simulink model "RobustFormationControl_IntegerModel_under_Dis"  (R2023a)
settings: Solver=ode3  StartTime=0.0  StopTime=30  FixedStep=0.0001  RelTol=1e-3
InitFcn:
  | % % Parameters for the fractional order NTFSMC:
  | % Sliding Surface " Sx, Sy, and Sz ":
  | %------------------------
  | % 10
  | % 10
  | cx = 2*[4 4 4];
  | cxx = 1*[0.01 0.01 0.01];
  | 
  | cx1 = cx(1);
  | cy1 = cx(2);
  | cz1 = cx(3);
  | 
  | cx2 = cxx(1);
  | cy2 = cxx(2);
  | cz2 = cxx(3);
  | 
  | alpha1 = [0.6 0.6 0.6];
  | alpha2 = [0.1 0.1 0.1];
  | 
  | gammaX = [3 3 3];
  | gx  = gammaX(1);
  | gy = gammaX(2);
  | gz = gammaX(3);
  | 
  | p = 10;
  | q = 10;
  | 
  | % Sliding Surface " S_Phi , S_Theta, and  S_Psi":
  | %------------------------
  | cP = 2*[4 4 4];
  | cPP = 1*[0.01 0.01 0.01 0.01];
  | 
  | cPhi1 = cP(1);
  | cTheta1 = cP(2);
  | cPsi1 = cP(3);
  | 
  | cPhi2 = cPP(1);
  | cTheta2 = cPP(2);
  | cPsi2 = cPP(3);
  | gammaP = [3 3 3];
  | 
  | %=========================
  | %=========================
  | SigmaX = 1*[0.01 0.01 0.01];
  | SigmaXX =1*[1 1 1];
  | 
  | Sigma1X = SigmaX(1);
  | Sigma1Y = SigmaX(2);
  | Sigma1Z = SigmaX(3);
  | %-----
  | Sigma2X = SigmaXX(1);
  | Sigma2Y = SigmaXX(2);
  | Sigma2Z = SigmaXX(3);
  | 
  | 
  | SigmaP = 1*[0.01 0.01 0.01];
  | SigmaPP =1*[1 1 1];
  | 
  | Sigma1Phi   = SigmaP(1);
  | Sigma1Theta = SigmaP(2);
  | ... (+80 lines)
values from neighbouring files (symbols this model uses):
  a1 = (Iyy - Izz)/Ixx    (= -0.812397034596)    [init_quadrotor_params.m]
  a2 = (Izz - Ixx)/Iyy    (= 0.812397034596)    [init_quadrotor_params.m]
  a3 = (Ixx - Iyy)/Izz    (= 0)    [init_quadrotor_params.m]
  a4 = - Ktx/m    (= -0.00114547325103)    [init_quadrotor_params.m]
  a5 = - Kty/m    (= -0.00114547325103)    [init_quadrotor_params.m]
  a6 = - Ktz/m    (= -0.00130740740741)    [init_quadrotor_params.m]
  b = 2.980e-5    (= 2.98e-05)    [init_quadrotor_params.m]
  b1 = - Jr/Ixx    (= -0.00584534596376)    [init_quadrotor_params.m]
  b2 = Jr/Iyy    (= 0.00584534596376)    [init_quadrotor_params.m]
  b3 = - Kfz/Izz    (= -0.0721963413248)    [init_quadrotor_params.m]
  b4 = 1/m    (= 2.05761316872)    [init_quadrotor_params.m]
  b5 = 1/m    (= 2.05761316872)    [init_quadrotor_params.m]
  b6 = 1/m    (= 2.05761316872)    [init_quadrotor_params.m]
  c1 = - Kfx/Ixx    (= -0.114641680395)    [init_quadrotor_params.m]
  c2 = - Kfy/Iyy    (= -0.114641680395)    [init_quadrotor_params.m]
  c3 = 1/Izz    (= 113.62345188)    [init_quadrotor_params.m]
  d = 1.12e-06    [init_quadrotor_params.m]
  d1 = L/Ixx    (= 46.334431631)    [init_quadrotor_params.m]
  d2 = L/Iyy    (= 46.334431631)    [init_quadrotor_params.m]
  g = 9.81    [init_quadrotor_params.m]
  Ixx = 4.856e-3    (= 0.004856)    [init_quadrotor_params.m]
  Iyy = 4.856e-3    (= 0.004856)    [init_quadrotor_params.m]
  Izz = 8.801e-3    (= 0.008801)    [init_quadrotor_params.m]
  Jr = 2.8385e-5    (= 2.8385e-05)    [init_quadrotor_params.m]
  Kfx = 5.567e-4    (= 0.0005567)    [init_quadrotor_params.m]
  Kfy = 5.567e-4    (= 0.0005567)    [init_quadrotor_params.m]
  Kfz = 6.354e-4    (= 0.0006354)    [init_quadrotor_params.m]
  Ktx = 5.5670e-4    (= 0.0005567)    [init_quadrotor_params.m]
  Kty = 5.5670e-4    (= 0.0005567)    [init_quadrotor_params.m]
  Ktz = 6.3540e-4    (= 0.0006354)    [init_quadrotor_params.m]
  L = 0.225    [init_quadrotor_params.m]
  m = 0.486    [init_quadrotor_params.m]
libraries: fod x120, eeStairGenerator x5
(part 2 of 9)

== system RobustFormationControl_IntegerModel_under_Dis/Integer Leader and four followers/Follower 3 System/ez ==
  note: error analysis for x - position
  note: error analysis for z - position
  note: error analysis for y - position
  e_x : Inport
  e_y : Inport  Port=2
  e_z : Inport  Port=3
  Abs : Abs  SaturateOnIntegerOverflow=off
  Abs1 : Abs  SaturateOnIntegerOverflow=off
  Abs2 : Abs  SaturateOnIntegerOverflow=off
  Clock1 : Clock
  IAE : Display
  IAE1 : Display
  IAE2 : Display
  ISE : Display
  ISE1 : Display
  ISE2 : Display
  ITAE : Display
  ITAE1 : Display
  ITAE2 : Display
  ITSE : Display
  ITSE1 : Display
  ITSE2 : Display
  Integrator{,1..11} (12 alike) : Integrator
  Math Function : Math  Operator=square
  Math Function1 : Math  Operator=square
  Math Function2 : Math  Operator=square
  Mux : Mux
  Mux1 : Mux
  Mux2 : Mux
  Product{,1..5} (6 alike) : Product
  To Workspace : ToWorkspace  VariableName=Ex3  SampleTime=-1
  To Workspace1 : ToWorkspace  VariableName=Ez3  SampleTime=-1
  To Workspace2 : ToWorkspace  VariableName=Ey3  SampleTime=-1
  wires:
  Abs/1 -> Product/1, Integrator/1
  Integrator/1 -> Mux/1, IAE/1
  Math Function/1 -> Product1/1, Integrator1/1
  Integrator1/1 -> Mux/2, ISE/1
  Product/1 -> Integrator2/1
  Integrator2/1 -> Mux/3, ITAE/1
  Product1/1 -> Integrator3/1
  Integrator3/1 -> Mux/4, ITSE/1
  [time] -> Product1/2, Product/2
  [time] -> Product2/2, Product3/2
  Integrator7/1 -> Mux2/4, ITSE1/1
  Product3/1 -> Integrator7/1
  Integrator6/1 -> Mux2/3, ITAE1/1
  Product2/1 -> Integrator6/1
  Integrator5/1 -> Mux2/2, ISE1/1
  Math Function1/1 -> Integrator5/1, Product3/1
  Integrator4/1 -> Mux2/1, IAE1/1
  Abs1/1 -> Integrator4/1, Product2/1
  [ey] -> Abs1/1, Math Function1/1
  [ez] -> Math Function2/1, Abs2/1
  Abs2/1 -> Product4/1, Integrator8/1
  Integrator8/1 -> Mux1/1, IAE2/1
  Math Function2/1 -> Product5/1, Integrator9/1
  Integrator9/1 -> Mux1/2, ISE2/1
  Product4/1 -> Integrator10/1
  Integrator10/1 -> Mux1/3, ITAE2/1
  Product5/1 -> Integrator11/1
  Integrator11/1 -> Mux1/4, ITSE2/1
  [time] -> Product5/2, Product4/2
  e_x/1 -> [ex]
  e_y/1 -> [ey]
  e_z/1 -> [ez]
  Clock1/1 -> [time]
  [ex] -> Math Function/1, Abs/1
  Mux/1 -> To Workspace/1
  Mux1/1 -> To Workspace1/1
  Mux2/1 -> To Workspace2/1

== system RobustFormationControl_IntegerModel_under_Dis/Integer Leader and four followers/Follower 4 System/Desired Values ==
  t : Inport
  Helical Trajectry : Subsystem  Commented=on
  Helical Trajectry1 : Subsystem
  Step : Step  Time=0  After=0.001  SampleTime=0
  Step Inputs Trajectry : Subsystem  Commented=on
  Phi_d : Outport  VectorParamsAs1DForOutWhenUnconnected=off
  Theta_d : Outport  Port=2  VectorParamsAs1DForOutWhenUnconnected=off
  Psi_d : Outport  Port=3  VectorParamsAs1DForOutWhenUnconnected=off
  Xd : Outport  Port=4  VectorParamsAs1DForOutWhenUnconnected=off
  Yd : Outport  Port=5  VectorParamsAs1DForOutWhenUnconnected=off
  Zd : Outport  Port=6  VectorParamsAs1DForOutWhenUnconnected=off
  wires:
  t/1 -> Helical Trajectry1/1(t), Helical Trajectry/1(t)
  Step/1 -> Theta_d/1, Phi_d/1
  Helical Trajectry1/1(xd) -> Xd/1
  Helical Trajectry1/4(Psi_d) -> Psi_d/1
  Helical Trajectry1/2(yd) -> Yd/1
  Helical Trajectry1/3(zd) -> Zd/1

== system RobustFormationControl_IntegerModel_under_Dis/Integer Leader and four followers/Follower 4 System/Follower 2 Quadrotor Model ==
  xd : Inport
  yd : Inport  Port=2
  zd : Inport  Port=3
  Psi_d : Inport  Port=4
  xLeader : Inport  Port=5
  dXYZ : Inport  Port=6
  Control Module1 : Subsystem
  Quadrotor Dynamic System : Subsystem
  X : Outport  VectorParamsAs1DForOutWhenUnconnected=off
  Y : Outport  Port=2  VectorParamsAs1DForOutWhenUnconnected=off
  Z : Outport  Port=3  VectorParamsAs1DForOutWhenUnconnected=off
  Phi : Outport  Port=4  VectorParamsAs1DForOutWhenUnconnected=off
  Theta : Outport  Port=5  VectorParamsAs1DForOutWhenUnconnected=off
  Psi : Outport  Port=6  VectorParamsAs1DForOutWhenUnconnected=off
  U1 : Outport  Port=7  VectorParamsAs1DForOutWhenUnconnected=off
  U2 : Outport  Port=8  VectorParamsAs1DForOutWhenUnconnected=off
  U3 : Outport  Port=9  VectorParamsAs1DForOutWhenUnconnected=off
  U4 : Outport  Port=10  VectorParamsAs1DForOutWhenUnconnected=off
  Ux : Outport  Port=11  VectorParamsAs1DForOutWhenUnconnected=off
  Uy : Outport  Port=12  VectorParamsAs1DForOutWhenUnconnected=off
  wires:
  Control Module1/5(Ux) -> Ux/1, Quadrotor Dynamic System/5(Ux)  "Ux"
  Quadrotor Dynamic System/2(y = x9) -> [x9], Y/1  "Y"
  Quadrotor Dynamic System/6(Psi) -> [x5], Psi/1  "Psi"
  Control Module1/4(U4) -> U4/1, Quadrotor Dynamic System/4(U4)  "U4"
  Quadrotor Dynamic System/3(z = x11) -> [x11], Z/1  "Z"
  Quadrotor Dynamic System/4(Phi) -> [x1], Phi/1  "Phi"
  Quadrotor Dynamic System/5(Theta) -> [x3], Theta/1  "Theta"
  Quadrotor Dynamic System/1(x = x7) -> [x7], X/1  "X"
  Control Module1/6(Uy) -> Uy/1, Quadrotor Dynamic System/6(Uy)  "Uy"
  Control Module1/1(U1) -> Quadrotor Dynamic System/1(U1), U1/1  "U1"
  Control Module1/2(U2) -> Quadrotor Dynamic System/2(U2), U2/1  "U2"
  Control Module1/3(U3) -> U3/1, Quadrotor Dynamic System/3(U3)  "U3"
  Control Module1/7(Omega) -> Quadrotor Dynamic System/7(Omega)
  Quadrotor Dynamic System/7(x2) -> [x2]
  Quadrotor Dynamic System/12(zdot = x12) -> [x12]
  Quadrotor Dynamic System/11(ydot = x10) -> [x10]
  Quadrotor Dynamic System/10(xdot = x8) -> [x8]
  Quadrotor Dynamic System/9(x6) -> [x6]
  Quadrotor Dynamic System/8(x4) -> [x4]
  [x1] -> Control Module1/1(x1)
  [x2] -> Control Module1/2(x2)
  [x3] -> Control Module1/3(x3)
  [x4] -> Control Module1/4(x4)
  [x5] -> Control Module1/5(x5)
  [x6] -> Control Module1/6(x6)
  [x7] -> Control Module1/7(x7)
  [x8] -> Control Module1/8(x8)
  [x9] -> Control Module1/9(x9)
  [x10] -> Control Module1/10(x10)
  [x11] -> Control Module1/11(x11)
  [x12] -> Control Module1/12(x12)
  xd/1 -> Control Module1/14(" xd")
  yd/1 -> Control Module1/15(yd)
  zd/1 -> Control Module1/16(" zd")
  Psi_d/1 -> Control Module1/13(Psi_d)
  xLeader/1 -> Control Module1/17(xLeader)
  dXYZ/1 -> Control Module1/18(Distance_d)

== system RobustFormationControl_IntegerModel_under_Dis/Integer Leader and four followers/Follower 4 System/Results Plot ==
  note: yL
  xF : Inport
  xL : Inport  Port=2
  Demux : Demux  Outputs=3
  Demux1 : Demux  Outputs=3
  x : Scope  NumInputPorts=2
  y : Scope  NumInputPorts=2
  z : Scope  NumInputPorts=2
  wires:
  xF/1 -> Demux/1
  xL/1 -> Demux1/1
  Demux/1 -> x/1  "xF"
  Demux1/1 -> x/2  "xL"
  Demux/2 -> y/1  "yF"
  Demux1/2 -> y/2
  Demux/3 -> z/1  "zF"
  Demux1/3 -> z/2  "zL"

== system RobustFormationControl_IntegerModel_under_Dis/Integer Leader and four followers/Follower 4 System/ez ==
  note: error analysis for x - position
  note: error analysis for z - position
  note: error analysis for y - position
  e_x : Inport
  e_y : Inport  Port=2
  e_z : Inport  Port=3
  Abs : Abs  SaturateOnIntegerOverflow=off
  Abs1 : Abs  SaturateOnIntegerOverflow=off
  Abs2 : Abs  SaturateOnIntegerOverflow=off
  Clock1 : Clock
  IAE : Display
  IAE1 : Display
  IAE2 : Display
  ISE : Display
  ISE1 : Display
  ISE2 : Display
  ITAE : Display
  ITAE1 : Display
  ITAE2 : Display
  ITSE : Display
  ITSE1 : Display
  ITSE2 : Display
  Integrator{,1..11} (12 alike) : Integrator
  Math Function : Math  Operator=square
  Math Function1 : Math  Operator=square
  Math Function2 : Math  Operator=square
  Mux : Mux
  Mux1 : Mux
  Mux2 : Mux
  Product{,1..5} (6 alike) : Product
  To Workspace : ToWorkspace  VariableName=Ex4  SampleTime=-1
  To Workspace1 : ToWorkspace  VariableName=Ez4  SampleTime=-1
  To Workspace2 : ToWorkspace  VariableName=Ey4  SampleTime=-1
  wires:
  Abs/1 -> Product/1, Integrator/1
  Integrator/1 -> Mux/1, IAE/1
  Math Function/1 -> Product1/1, Integrator1/1
  Integrator1/1 -> Mux/2, ISE/1
  Product/1 -> Integrator2/1
  Integrator2/1 -> Mux/3, ITAE/1
  Product1/1 -> Integrator3/1
  Integrator3/1 -> Mux/4, ITSE/1
  [time] -> Product1/2, Product/2
  [time] -> Product2/2, Product3/2
  Integrator7/1 -> Mux2/4, ITSE1/1
  Product3/1 -> Integrator7/1
  Integrator6/1 -> Mux2/3, ITAE1/1
  Product2/1 -> Integrator6/1
  Integrator5/1 -> Mux2/2, ISE1/1
  Math Function1/1 -> Integrator5/1, Product3/1
  Integrator4/1 -> Mux2/1, IAE1/1
  Abs1/1 -> Integrator4/1, Product2/1
  [ey] -> Abs1/1, Math Function1/1
  [ez] -> Math Function2/1, Abs2/1
  Abs2/1 -> Product4/1, Integrator8/1
  Integrator8/1 -> Mux1/1, IAE2/1
  Math Function2/1 -> Product5/1, Integrator9/1
  Integrator9/1 -> Mux1/2, ISE2/1
  Product4/1 -> Integrator10/1
  Integrator10/1 -> Mux1/3, ITAE2/1
  Product5/1 -> Integrator11/1
  Integrator11/1 -> Mux1/4, ITSE2/1
  [time] -> Product5/2, Product4/2
  e_x/1 -> [ex]
  e_y/1 -> [ey]
  e_z/1 -> [ez]
  Clock1/1 -> [time]
  [ex] -> Math Function/1, Abs/1
  Mux/1 -> To Workspace/1
  Mux1/1 -> To Workspace1/1
  Mux2/1 -> To Workspace2/1

== system RobustFormationControl_IntegerModel_under_Dis/Integer Leader and four followers/Leader System/Desired Values ==
  t : Inport
  Circular Trajectry : Subsystem  Commented=on
  Helical Trajectry : Subsystem
  Step : Step  Time=0  After=0.001  SampleTime=0
  Step Inputs Trajectry : Subsystem  Commented=on
  Phi_d : Outport  VectorParamsAs1DForOutWhenUnconnected=off
  Theta_d : Outport  Port=2  VectorParamsAs1DForOutWhenUnconnected=off
  Psi_d : Outport  Port=3  VectorParamsAs1DForOutWhenUnconnected=off
  Xd : Outport  Port=4  VectorParamsAs1DForOutWhenUnconnected=off
  Yd : Outport  Port=5  VectorParamsAs1DForOutWhenUnconnected=off
  Zd : Outport  Port=6  VectorParamsAs1DForOutWhenUnconnected=off
  wires:
  t/1 -> Circular Trajectry/1(t), Helical Trajectry/1(t)
  Step/1 -> Theta_d/1, Phi_d/1
  Helical Trajectry/3(zd) -> Zd/1
  Helical Trajectry/2(yd) -> Yd/1
  Helical Trajectry/1(xd) -> Xd/1
  Helical Trajectry/4(Psi_d) -> Psi_d/1

== system RobustFormationControl_IntegerModel_under_Dis/Integer Leader and four followers/Leader System/Integer Model ==
  xd : Inport
  yd : Inport  Port=2
  zd : Inport  Port=3
  Psi_d : Inport  Port=4
  Control Module1 : Subsystem
  Quadrotor Dynamic System : Subsystem
  Scope : Scope
  X : Outport  VectorParamsAs1DForOutWhenUnconnected=off
  Y : Outport  Port=2  VectorParamsAs1DForOutWhenUnconnected=off
  Z : Outport  Port=3  VectorParamsAs1DForOutWhenUnconnected=off
  Phi : Outport  Port=4  VectorParamsAs1DForOutWhenUnconnected=off
  Theta : Outport  Port=5  VectorParamsAs1DForOutWhenUnconnected=off
  Psi : Outport  Port=6  VectorParamsAs1DForOutWhenUnconnected=off
  U1 : Outport  Port=7  VectorParamsAs1DForOutWhenUnconnected=off
  U2 : Outport  Port=8  VectorParamsAs1DForOutWhenUnconnected=off
  U3 : Outport  Port=9  VectorParamsAs1DForOutWhenUnconnected=off
  U4 : Outport  Port=10  VectorParamsAs1DForOutWhenUnconnected=off
  Ux : Outport  Port=11  VectorParamsAs1DForOutWhenUnconnected=off
  Uy : Outport  Port=12  VectorParamsAs1DForOutWhenUnconnected=off
  wires:
  Control Module1/5(Ux) -> Ux/1, Quadrotor Dynamic System/5(Ux)  "Ux"
  Quadrotor Dynamic System/2(y = x9) -> [x9], Y/1  "Y"
  Quadrotor Dynamic System/6(Psi) -> [x5], Psi/1  "Psi"
  Control Module1/4(U4) -> U4/1, Quadrotor Dynamic System/4(U4)  "U4"
  Quadrotor Dynamic System/3(z = x11) -> [x11], Z/1  "Z"
  Quadrotor Dynamic System/4(Phi) -> [x1], Scope/1, Phi/1  "Phi"
  Quadrotor Dynamic System/5(Theta) -> [x3], Theta/1  "Theta"
  Quadrotor Dynamic System/1(x = x7) -> [x7], X/1  "X"
  Control Module1/6(Uy) -> Uy/1, Quadrotor Dynamic System/6(Uy)  "Uy"
  Control Module1/1(U1) -> Quadrotor Dynamic System/1(U1), U1/1  "U1"
  Control Module1/2(U2) -> Quadrotor Dynamic System/2(U2), U2/1  "U2"
  Control Module1/3(U3) -> U3/1, Quadrotor Dynamic System/3(U3)  "U3"
  Control Module1/7(Omega) -> Quadrotor Dynamic System/7(Omega)
  Quadrotor Dynamic System/7(x2) -> [x2]
  Quadrotor Dynamic System/12(zdot = x12) -> [x12]
  Quadrotor Dynamic System/11(ydot = x10) -> [x10]
  Quadrotor Dynamic System/10(xdot = x8) -> [x8]
  Quadrotor Dynamic System/9(x6) -> [x6]
  Quadrotor Dynamic System/8(x4) -> [x4]
  [x1] -> Control Module1/1(x1)
  [x2] -> Control Module1/2(x2)
  [x3] -> Control Module1/3(x3)
  [x4] -> Control Module1/4(x4)
  [x5] -> Control Module1/5(x5)
  [x6] -> Control Module1/6(x6)
  [x7] -> Control Module1/7(x7)
  [x8] -> Control Module1/8(x8)
  [x9] -> Control Module1/9(x9)
  [x10] -> Control Module1/10(x10)
  [x11] -> Control Module1/11(x11)
  [x12] -> Control Module1/12(x12)
  xd/1 -> Control Module1/14(" xd")
  yd/1 -> Control Module1/15(yd)
  zd/1 -> Control Module1/16(" zd")
  Psi_d/1 -> Control Module1/13(Psi_d)

== system RobustFormationControl_IntegerModel_under_Dis/Integer Leader and four followers/Leader System/Stochastic Disturbances ==
  Dphi1 : Subsystem
  Dphi2 : Subsystem
  Dphi3 : Subsystem
  Dpx : Subsystem
  Dpy : Subsystem
  Dpz : Subsystem
  Mux : Mux  Inputs=3
  Mux1 : Mux  Inputs=3
  To Workspace : ToWorkspace  VariableName=DisP  SampleTime=-1
  To Workspace1 : ToWorkspace  VariableName=DisA  SampleTime=-1
  tag scope: Dphi1=global, Dphi2=global, Dphi3=global, Dpx=global, Dpy=global, Dpz=global
  wires:
  Dpx/1(Dpx) -> [Dpx]
  Dpy/1(Dpy) -> [Dpy]
  Dpz/1(Dpz) -> [Dpz]
  Dphi1/1(Dphi1) -> [Dphi1]
  Dphi2/1(Dphi2) -> [Dphi2]
  Dphi3/1(Dphi3) -> [Dphi3]
  Mux/1 -> To Workspace/1
  Mux1/1 -> To Workspace1/1
  [Dpx] -> Mux/1
  [Dpy] -> Mux/2
  [Dpz] -> Mux/3
  [Dphi1] -> Mux1/1
  [Dphi2] -> Mux1/2
  [Dphi3] -> Mux1/3

== system RobustFormationControl_IntegerModel_under_Dis/Integer Leader and four followers/Leader System/Uncertainity ==
  uncertainity in mass : Subsystem
  uncertainity in moments of inertia : Subsystem

== system RobustFormationControl_IntegerModel_under_Dis/Integer Leader and four followers/Leader System/ez ==
  note: error analysis for x - position
  note: error analysis for z - position
  note: error analysis for y - position
  e_x : Inport
  e_y : Inport  Port=2
  e_z : Inport  Port=3
  Abs : Abs  SaturateOnIntegerOverflow=off
  Abs1 : Abs  SaturateOnIntegerOverflow=off
  Abs2 : Abs  SaturateOnIntegerOverflow=off
  Clock1 : Clock
  IAE : Display
  IAE1 : Display
  IAE2 : Display
  ISE : Display
  ISE1 : Display
  ISE2 : Display
  ITAE : Display
  ITAE1 : Display
  ITAE2 : Display
  ITSE : Display
  ITSE1 : Display
  ITSE2 : Display
  Integrator{,1..11} (12 alike) : Integrator
  Math Function : Math  Operator=square
  Math Function1 : Math  Operator=square
  Math Function2 : Math  Operator=square
  Mux : Mux
  Mux1 : Mux
  Mux2 : Mux
  Product{,1..5} (6 alike) : Product
  To Workspace : ToWorkspace  VariableName=Ex  SampleTime=-1
  To Workspace1 : ToWorkspace  VariableName=Ez  SampleTime=-1
  To Workspace2 : ToWorkspace  VariableName=Ey  SampleTime=-1
  wires:
  Abs/1 -> Product/1, Integrator/1
  Integrator/1 -> Mux/1, IAE/1
  Math Function/1 -> Product1/1, Integrator1/1
  Integrator1/1 -> Mux/2, ISE/1
  Product/1 -> Integrator2/1
  Integrator2/1 -> Mux/3, ITAE/1
  Product1/1 -> Integrator3/1
  Integrator3/1 -> Mux/4, ITSE/1
  [time] -> Product1/2, Product/2
  [time] -> Product2/2, Product3/2
  Integrator7/1 -> Mux2/4, ITSE1/1
  Product3/1 -> Integrator7/1
  Integrator6/1 -> Mux2/3, ITAE1/1
  Product2/1 -> Integrator6/1
  Integrator5/1 -> Mux2/2, ISE1/1
  Math Function1/1 -> Integrator5/1, Product3/1
  Integrator4/1 -> Mux2/1, IAE1/1
  Abs1/1 -> Integrator4/1, Product2/1
  [ey] -> Abs1/1, Math Function1/1
  [ez] -> Math Function2/1, Abs2/1
  Abs2/1 -> Product4/1, Integrator8/1
  Integrator8/1 -> Mux1/1, IAE2/1
  Math Function2/1 -> Product5/1, Integrator9/1
  Integrator9/1 -> Mux1/2, ISE2/1
  Product4/1 -> Integrator10/1
  Integrator10/1 -> Mux1/3, ITAE2/1
  Product5/1 -> Integrator11/1
  Integrator11/1 -> Mux1/4, ITSE2/1
  [time] -> Product5/2, Product4/2
  e_x/1 -> [ex]
  e_y/1 -> [ey]
  e_z/1 -> [ez]
  Clock1/1 -> [time]
  [ex] -> Math Function/1, Abs/1
  Mux/1 -> To Workspace/1
  Mux1/1 -> To Workspace1/1
  Mux2/1 -> To Workspace2/1

== system RobustFormationControl_IntegerModel_under_Dis/Integer Leader and four followers/Follower 1 System/Desired Values/Helical Trajectry ==
  t : Inport
  Gain2 : Gain  Gain=0.2
  Step1 : Step  Time=0  SampleTime=0
  Trigonometric Function : Trigonometry
  Trigonometric Function1 : Trigonometry  Operator=cos
  xd : Outport  VectorParamsAs1DForOutWhenUnconnected=off
  yd : Outport  Port=2  VectorParamsAs1DForOutWhenUnconnected=off
  zd : Outport  Port=3  VectorParamsAs1DForOutWhenUnconnected=off
  Psi_d : Outport  Port=4  VectorParamsAs1DForOutWhenUnconnected=off
  wires:
  t/1 -> Trigonometric Function1/1, Trigonometric Function/1, Gain2/1
  Gain2/1 -> zd/1
  Step1/1 -> Psi_d/1
  Trigonometric Function1/1 -> xd/1
  Trigonometric Function/1 -> yd/1

== system RobustFormationControl_IntegerModel_under_Dis/Integer Leader and four followers/Follower 1 System/Desired Values/Helical Trajectry1 ==
  t : Inport
  Gain : Gain  Gain=dis
  Gain1 : Gain  Gain=2*pi/15
  Gain2 : Gain  Gain=1/15
  Gain3 : Gain  Gain=2*pi/15
  Scope : Scope
  Step : Step  Time=0  After=0  SampleTime=0.03
  Step1 : Step  Time=0  SampleTime=0
  Step2 : Step  Time=5  After=0.5  SampleTime=0.03
  Step3 : Step  Time=10  After=0.5  SampleTime=0.03
  Sum : Sum  Inputs=++-
  Sum1 : Sum  Inputs=|++
  Trigonometric Function : Trigonometry  Operator=cos
  Trigonometric Function1 : Trigonometry
  xd : Outport  VectorParamsAs1DForOutWhenUnconnected=off
  yd : Outport  Port=2  VectorParamsAs1DForOutWhenUnconnected=off
  zd : Outport  Port=3  VectorParamsAs1DForOutWhenUnconnected=off
  Psi_d : Outport  Port=4  VectorParamsAs1DForOutWhenUnconnected=off
  wires:
  t/1 -> Gain1/1, Gain3/1, Gain2/1
  Gain2/1 -> zd/1
  Step1/1 -> Psi_d/1
  Trigonometric Function1/1 -> yd/1
  Step/1 -> Sum/1
  Sum/1 -> Gain/1, Scope/1
  Step2/1 -> Sum/2
  Step3/1 -> Sum/3
  Sum1/1 -> xd/1
  Trigonometric Function/1 -> Sum1/2
  Gain/1 -> Sum1/1
  Gain1/1 -> Trigonometric Function/1
  Gain3/1 -> Trigonometric Function1/1

== system RobustFormationControl_IntegerModel_under_Dis/Integer Leader and four followers/Follower 1 System/Desired Values/Step Inputs Trajectry ==
  Step : Step  Time=0  After=3  SampleTime=0
  Step1 : Step  Time=0  After=5  SampleTime=0
  Step2 : Step  Time=0  SampleTime=0
  Step3 : Step  Time=0  After=2  SampleTime=0
  xd : Outport  VectorParamsAs1DForOutWhenUnconnected=off
  yd : Outport  Port=2  VectorParamsAs1DForOutWhenUnconnected=off
  zd : Outport  Port=3  VectorParamsAs1DForOutWhenUnconnected=off
  Psi_d : Outport  Port=4  VectorParamsAs1DForOutWhenUnconnected=off
  wires:
  Step2/1 -> xd/1
  Step3/1 -> yd/1
  Step/1 -> zd/1
  Step1/1 -> Psi_d/1

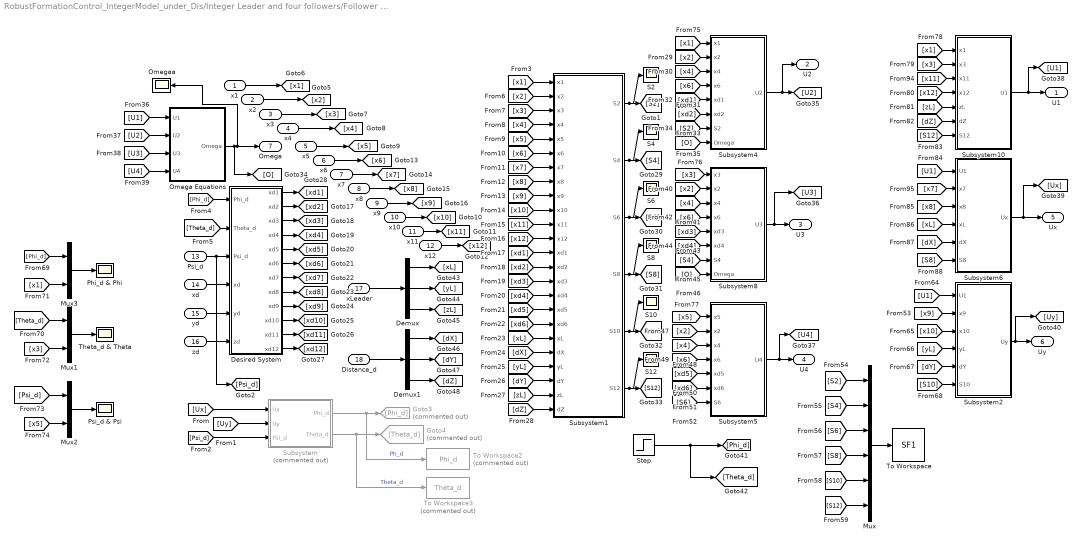
== system RobustFormationControl_IntegerModel_under_Dis/Integer Leader and four followers/Follower 1 System/Follower 1 Quadrotor Model/Control Module1 ==
  x1 : Inport
  x2 : Inport  Port=2
  x3 : Inport  Port=3
  x4 : Inport  Port=4
  x5 : Inport  Port=5
  x6 : Inport  Port=6
  x7 : Inport  Port=7
  x8 : Inport  Port=8
  x9 : Inport  Port=9
  x10 : Inport  Port=10
  x11 : Inport  Port=11
  x12 : Inport  Port=12
  Psi_d : Inport  Port=13
  " xd" : Inport  Port=14
  yd : Inport  Port=15
  " zd" : Inport  Port=16
  xLeader : Inport  Port=17
  Distance_d : Inport  Port=18
  " Phi_d & Phi" : Scope
  " Theta_d & Theta" : Scope
  Demux : Demux  Outputs=3
  Demux1 : Demux  Outputs=3
  Desired System : Subsystem
  Goto3 : Goto  Commented=on  GotoTag=Phi_d
  Goto4 : Goto  Commented=on  GotoTag=Theta_d
  Mux : Mux  Inputs=6
  Mux1 : Mux  Inputs=2
  Mux2 : Mux  Inputs=2
  Mux3 : Mux  Inputs=2
  Omega Equations : Subsystem
  Omegaa : Scope
  Psi_d & Psi : Scope
  S{4,6,8,10,12} (5 alike) : Scope
  "S2 " : Scope
  Step : Step  Time=0  After=0.001  SampleTime=0
  Subsystem : Subsystem  Commented=on
  Subsystem1 : Subsystem
  Subsystem10 : Subsystem
  Subsystem2 : Subsystem
  Subsystem4 : Subsystem
  Subsystem5 : Subsystem
  Subsystem6 : Subsystem
  Subsystem8 : Subsystem
  To Workspace : ToWorkspace  VariableName=SF1  SampleTime=-1
  To Workspace2 : ToWorkspace  Commented=on  VariableName=Phi_d  SampleTime=-1
  To Workspace3 : ToWorkspace  Commented=on  VariableName=Theta_d  SampleTime=-1
  U1 : Outport  VectorParamsAs1DForOutWhenUnconnected=off
  U2 : Outport  Port=2  VectorParamsAs1DForOutWhenUnconnected=off
  U3 : Outport  Port=3  VectorParamsAs1DForOutWhenUnconnected=off
  U4 : Outport  Port=4  VectorParamsAs1DForOutWhenUnconnected=off
  Ux : Outport  Port=5  VectorParamsAs1DForOutWhenUnconnected=off
  Uy : Outport  Port=6  VectorParamsAs1DForOutWhenUnconnected=off
  Omega : Outport  Port=7  VectorParamsAs1DForOutWhenUnconnected=off
  wires:
  Omega Equations/1(Omega) -> [O], Omegaa/1, Omega/1
  [Ux] -> Subsystem/1(Ux)
  [Uy] -> Subsystem/2(Uy)
  [Psi_d] -> Subsystem/3(Psi_d)
  Subsystem/1(Phi_d) -> To Workspace2/1, Goto3/1  "Ph_d"
  Subsystem/2(Theta_d) -> To Workspace3/1, Goto4/1  "Theta_d"
  [xd1] -> Subsystem1/13(xd1)
  [xd2] -> Subsystem1/14(xd2)
  [xd3] -> Subsystem1/15(xd3)
  [xd4] -> Subsystem1/16(xd4)
  [xd5] -> Subsystem1/17(xd5)
  [xd6] -> Subsystem1/18(xd6)
  [xL] -> Subsystem1/19(xL)
  [dX] -> Subsystem1/20(dX)
  [yL] -> Subsystem1/21(yL)
  [dY] -> Subsystem1/22(dY)
  [zL] -> Subsystem1/23(zL)
  [dZ] -> Subsystem1/24(dZ)
  x9/1 -> [x9]
  x5/1 -> [x5]
  x6/1 -> [x6]
  x1/1 -> [x1]
  x4/1 -> [x4]
  x3/1 -> [x3]
  x11/1 -> [x11]
  x10/1 -> [x10]
  x8/1 -> [x8]
  x2/1 -> [x2]
  x7/1 -> [x7]
  x12/1 -> [x12]
  [Phi_d] -> Desired System/1(Phi_d)
  [Theta_d] -> Desired System/2(Theta_d)
  Psi_d/1 -> [Psi_d], Desired System/3(Psi_d)
  " xd"/1 -> Desired System/4(xd)
  yd/1 -> Desired System/5(yd)
  Desired System/2(xd2) -> [xd2]
  Desired System/3(xd3) -> [xd3]
  Desired System/4(xd4) -> [xd4]
  Desired System/5(xd5) -> [xd5]
  Desired System/6(xd6) -> [xd6]
  Desired System/7(xd7) -> [xd7]
  Desired System/8(xd8) -> [xd8]
  Desired System/9(xd9) -> [xd9]
  Desired System/10(xd10) -> [xd10]
  Desired System/11(xd11) -> [xd11]
  Desired System/12(xd12) -> [xd12]
  Desired System/1(xd1) -> [xd1]
  " zd"/1 -> Desired System/6(zd)
  [x1] -> Subsystem1/1(x1)
  [x12] -> Subsystem1/12(x12)
  [x11] -> Subsystem1/11(x11)
  [x10] -> Subsystem1/10(x10)
  [x9] -> Subsystem1/9(x9)
  [x8] -> Subsystem1/8(x8)
  [x7] -> Subsystem1/7(x7)
  [x6] -> Subsystem1/6(x6)
  [x5] -> Subsystem1/5(x5)
  [x4] -> Subsystem1/4(x4)
  [x3] -> Subsystem1/3(x3)
  [x2] -> Subsystem1/2(x2)
  Subsystem1/1(S2) -> "S2 "/1, [S2]
  Subsystem1/2(S4) -> S4/1, [S4]
  Subsystem1/3(S6) -> S6/1, [S6]
  Subsystem1/4(S8) -> S8/1, [S8]
  Subsystem1/5(S10) -> S10/1, [S10]
  Subsystem1/6(S12) -> S12/1, [S12]
  [U1] -> Omega Equations/1(U1)
  [U4] -> Omega Equations/4(U4)
  [U3] -> Omega Equations/3(U3)
  [U2] -> Omega Equations/2(U2)
  Step/1 -> [Theta_d], [Phi_d]
  Mux3/1 -> " Phi_d & Phi"/1
  Mux1/1 -> " Theta_d & Theta"/1
  [Phi_d] -> Mux3/1
  [Theta_d] -> Mux1/1
  [x1] -> Mux3/2
  [x3] -> Mux1/2
  Mux2/1 -> Psi_d & Psi/1
  [Psi_d] -> Mux2/1
  [x5] -> Mux2/2
  Demux/1 -> [xL]
  Demux/2 -> [yL]
  Demux/3 -> [zL]
  Demux1/2 -> [dY]
  Demux1/3 -> [dZ]
  Demux1/1 -> [dX]
  xLeader/1 -> Demux/1
  Distance_d/1 -> Demux1/1
  [x2] -> Subsystem4/2(x2)
  [O] -> Subsystem4/8(Omega)
  [x6] -> Subsystem4/4(x6)
  [xd4] -> Subsystem8/6(xd4)
  [xd2] -> Subsystem4/6(xd2)
  [x3] -> Subsystem8/1(x3)
  Subsystem8/1(U3) -> [U3], U3/1
  Subsystem4/1(U2) -> U2/1, [U2]
  [x1] -> Subsystem4/1(x1)
  [x5] -> Subsystem5/1(x5)
  [O] -> Subsystem8/8(Omega)
  [x6] -> Subsystem5/4(x6)
  [S2] -> Subsystem4/7(S2)
  [xd3] -> Subsystem8/5(xd3)
  [S6] -> Subsystem5/7(S6)
  [xd1] -> Subsystem4/5(xd1)
  Subsystem5/1(U4) -> [U4], U4/1
  [x2] -> Subsystem5/2(x2)
  [x6] -> Subsystem8/4(x6)
  [xd6] -> Subsystem5/6(xd6)
  [x2] -> Subsystem8/2(x2)
  [S4] -> Subsystem8/7(S4)
  [x4] -> Subsystem8/3(x4)
  [xd5] -> Subsystem5/5(xd5)
  [x4] -> Subsystem4/3(x4)
  [x4] -> Subsystem5/3(x4)
  Subsystem10/1(U1) -> [U1], U1/1
  [x12] -> Subsystem10/4(x12)
  [x11] -> Subsystem10/3(x11)
  [dZ] -> Subsystem10/6(dZ)
  [S12] -> Subsystem10/7(S12)
  Subsystem6/1(Ux) -> [Ux], Ux/1
  [x1] -> Subsystem10/1(x1)
  [dX] -> Subsystem6/5(dX)
  [zL] -> Subsystem10/5(zL)
  [S8] -> Subsystem6/6(S8)
  [xL] -> Subsystem6/4(xL)
  [x8] -> Subsystem6/3(x8)
  [x7] -> Subsystem6/2(x7)
  [x3] -> Subsystem10/2(x3)
  [U1] -> Subsystem6/1(U1)
  Subsystem2/1(Uy) -> [Uy], Uy/1
  [U1] -> Subsystem2/1(U1)
  [x10] -> Subsystem2/3(x10)
  [yL] -> Subsystem2/4(yL)
  [S10] -> Subsystem2/6(S10)
  [dY] -> Subsystem2/5(dY)
  [x9] -> Subsystem2/2(x9)
  [S10] -> Mux/5
  [S6] -> Mux/3
  [S8] -> Mux/4
  [S2] -> Mux/1
  Mux/1 -> To Workspace/1
  [S4] -> Mux/2
  [S12] -> Mux/6

== system RobustFormationControl_IntegerModel_under_Dis/Integer Leader and four followers/Follower 1 System/Follower 1 Quadrotor Model/Quadrotor Dynamic System ==
  U1 : Inport
  U2 : Inport  Port=2
  U3 : Inport  Port=3
  U4 : Inport  Port=4
  Ux : Inport  Port=5
  Uy : Inport  Port=6
  Omega : Inport  Port=7
  Rotational System : Subsystem
  Translational System : Subsystem
  x = x7 : Outport  VectorParamsAs1DForOutWhenUnconnected=off
  y = x9 : Outport  Port=2  VectorParamsAs1DForOutWhenUnconnected=off
  z = x11 : Outport  Port=3  VectorParamsAs1DForOutWhenUnconnected=off
  Phi : Outport  Port=4  VectorParamsAs1DForOutWhenUnconnected=off
  Theta : Outport  Port=5  VectorParamsAs1DForOutWhenUnconnected=off
  Psi : Outport  Port=6  VectorParamsAs1DForOutWhenUnconnected=off
  x2 : Outport  Port=7  VectorParamsAs1DForOutWhenUnconnected=off
  x4 : Outport  Port=8  VectorParamsAs1DForOutWhenUnconnected=off
  x6 : Outport  Port=9  VectorParamsAs1DForOutWhenUnconnected=off
  xdot = x8 : Outport  Port=10  VectorParamsAs1DForOutWhenUnconnected=off
  ydot = x10 : Outport  Port=11  VectorParamsAs1DForOutWhenUnconnected=off
  zdot = x12 : Outport  Port=12  VectorParamsAs1DForOutWhenUnconnected=off
  wires:
  Rotational System/2(Theta or x3) -> Translational System/5(x3), Theta/1  "Theta"
  Rotational System/1(Phi or x1) -> Translational System/4(x1), Phi/1  "Phi"
  U4/1 -> Rotational System/3(U4)
  U2/1 -> Rotational System/1(U2)
  U3/1 -> Rotational System/2(U3)
  Rotational System/3(Psi or x5) -> Psi/1  "Psi"
  Translational System/3(z or x11) -> z = x11/1  "Z"
  Omega/1 -> Rotational System/4(Omega)
  U1/1 -> Translational System/1(U1)
  Translational System/2(y or x9) -> y = x9/1  "Y"
  Translational System/1(x or x7) -> x = x7/1  "X"
  Ux/1 -> Translational System/2(Ux)
  Uy/1 -> Translational System/3(Uy)
  Translational System/4(xdot or x8) -> xdot = x8/1
  Translational System/5(ydot or x10) -> ydot = x10/1
  Translational System/6(zdot or x12) -> zdot = x12/1
  Rotational System/4(x2) -> x2/1
  Rotational System/5(x4) -> x4/1
  Rotational System/6(x6) -> x6/1

== system RobustFormationControl_IntegerModel_under_Dis/Integer Leader and four followers/Follower 2 System/Desired Values/Helical Trajectry ==
  t : Inport
  Gain2 : Gain  Gain=0.2
  Step1 : Step  Time=0  SampleTime=0
  Trigonometric Function : Trigonometry
  Trigonometric Function1 : Trigonometry  Operator=cos
  xd : Outport  VectorParamsAs1DForOutWhenUnconnected=off
  yd : Outport  Port=2  VectorParamsAs1DForOutWhenUnconnected=off
  zd : Outport  Port=3  VectorParamsAs1DForOutWhenUnconnected=off
  Psi_d : Outport  Port=4  VectorParamsAs1DForOutWhenUnconnected=off
  wires:
  t/1 -> Trigonometric Function1/1, Trigonometric Function/1, Gain2/1
  Gain2/1 -> zd/1
  Step1/1 -> Psi_d/1
  Trigonometric Function1/1 -> xd/1
  Trigonometric Function/1 -> yd/1

== system RobustFormationControl_IntegerModel_under_Dis/Integer Leader and four followers/Follower 2 System/Desired Values/Helical Trajectry1 ==
  t : Inport
  Gain : Gain  Gain=dis
  Gain1 : Gain  Gain=2*pi/15
  Gain2 : Gain  Gain=1/15
  Gain3 : Gain  Gain=2*pi/15
  Scope : Scope
  Step : Step  Time=0  After=0  SampleTime=0.03
  Step1 : Step  Time=0  SampleTime=0
  Step2 : Step  Time=5  After=0.5  SampleTime=0.03
  Step3 : Step  Time=10  After=0.5  SampleTime=0.03
  Sum : Sum  Inputs=++-
  Sum1 : Sum  Inputs=|++
  Trigonometric Function : Trigonometry  Operator=cos
  Trigonometric Function1 : Trigonometry
  xd : Outport  VectorParamsAs1DForOutWhenUnconnected=off
  yd : Outport  Port=2  VectorParamsAs1DForOutWhenUnconnected=off
  zd : Outport  Port=3  VectorParamsAs1DForOutWhenUnconnected=off
  Psi_d : Outport  Port=4  VectorParamsAs1DForOutWhenUnconnected=off
  wires:
  t/1 -> Gain1/1, Gain3/1, Gain2/1
  Gain2/1 -> zd/1
  Step1/1 -> Psi_d/1
  Trigonometric Function1/1 -> yd/1
  Step/1 -> Sum/1
  Sum/1 -> Gain/1, Scope/1
  Step2/1 -> Sum/2
  Step3/1 -> Sum/3
  Sum1/1 -> xd/1
  Trigonometric Function/1 -> Sum1/2
  Gain/1 -> Sum1/1
  Gain1/1 -> Trigonometric Function/1
  Gain3/1 -> Trigonometric Function1/1

== system RobustFormationControl_IntegerModel_under_Dis/Integer Leader and four followers/Follower 2 System/Desired Values/Step Inputs Trajectry ==
  Step : Step  Time=0  After=3  SampleTime=0
  Step1 : Step  Time=0  After=5  SampleTime=0
  Step2 : Step  Time=0  SampleTime=0
  Step3 : Step  Time=0  After=2  SampleTime=0
  xd : Outport  VectorParamsAs1DForOutWhenUnconnected=off
  yd : Outport  Port=2  VectorParamsAs1DForOutWhenUnconnected=off
  zd : Outport  Port=3  VectorParamsAs1DForOutWhenUnconnected=off
  Psi_d : Outport  Port=4  VectorParamsAs1DForOutWhenUnconnected=off
  wires:
  Step2/1 -> xd/1
  Step3/1 -> yd/1
  Step/1 -> zd/1
  Step1/1 -> Psi_d/1

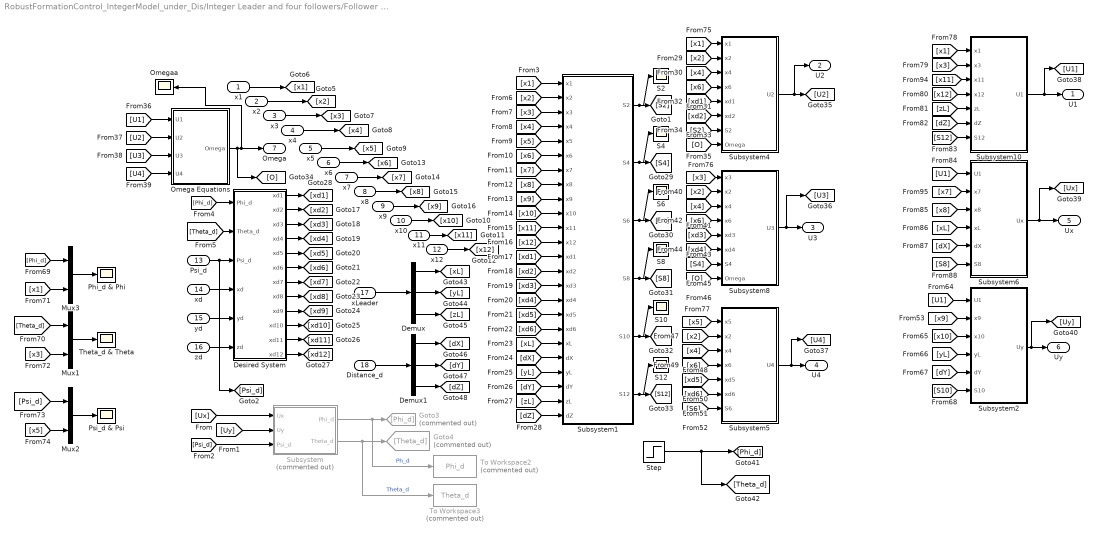
== system RobustFormationControl_IntegerModel_under_Dis/Integer Leader and four followers/Follower 2 System/Follower 2 Quadrotor Model/Control Module1 ==
  x1 : Inport
  x2 : Inport  Port=2
  x3 : Inport  Port=3
  x4 : Inport  Port=4
  x5 : Inport  Port=5
  x6 : Inport  Port=6
  x7 : Inport  Port=7
  x8 : Inport  Port=8
  x9 : Inport  Port=9
  x10 : Inport  Port=10
  x11 : Inport  Port=11
  x12 : Inport  Port=12
  Psi_d : Inport  Port=13
  " xd" : Inport  Port=14
  yd : Inport  Port=15
  " zd" : Inport  Port=16
  xLeader : Inport  Port=17
  Distance_d : Inport  Port=18
  " Phi_d & Phi" : Scope
  " Theta_d & Theta" : Scope
  Demux : Demux  Outputs=3
  Demux1 : Demux  Outputs=3
  Desired System : Subsystem
  Goto3 : Goto  Commented=on  GotoTag=Phi_d
  Goto4 : Goto  Commented=on  GotoTag=Theta_d
  Mux1 : Mux  Inputs=2
  Mux2 : Mux  Inputs=2
  Mux3 : Mux  Inputs=2
  Omega Equations : Subsystem
  Omegaa : Scope
  Psi_d & Psi : Scope
  S{4,6,8,10,12} (5 alike) : Scope
  "S2 " : Scope
  Step : Step  Time=0  After=0.001  SampleTime=0
  Subsystem : Subsystem  Commented=on
  Subsystem1 : Subsystem
  Subsystem10 : Subsystem
  Subsystem2 : Subsystem
  Subsystem4 : Subsystem
  Subsystem5 : Subsystem
  Subsystem6 : Subsystem
  Subsystem8 : Subsystem
  To Workspace2 : ToWorkspace  Commented=on  VariableName=Phi_d  SampleTime=-1
  To Workspace3 : ToWorkspace  Commented=on  VariableName=Theta_d  SampleTime=-1
  U1 : Outport  VectorParamsAs1DForOutWhenUnconnected=off
  U2 : Outport  Port=2  VectorParamsAs1DForOutWhenUnconnected=off
  U3 : Outport  Port=3  VectorParamsAs1DForOutWhenUnconnected=off
  U4 : Outport  Port=4  VectorParamsAs1DForOutWhenUnconnected=off
  Ux : Outport  Port=5  VectorParamsAs1DForOutWhenUnconnected=off
  Uy : Outport  Port=6  VectorParamsAs1DForOutWhenUnconnected=off
  Omega : Outport  Port=7  VectorParamsAs1DForOutWhenUnconnected=off
  wires:
  Omega Equations/1(Omega) -> [O], Omegaa/1, Omega/1
  [Ux] -> Subsystem/1(Ux)
  [Uy] -> Subsystem/2(Uy)
  [Psi_d] -> Subsystem/3(Psi_d)
  Subsystem/1(Phi_d) -> To Workspace2/1, Goto3/1  "Ph_d"
  Subsystem/2(Theta_d) -> To Workspace3/1, Goto4/1  "Theta_d"
  [xd1] -> Subsystem1/13(xd1)
  [xd2] -> Subsystem1/14(xd2)
  [xd3] -> Subsystem1/15(xd3)
  [xd4] -> Subsystem1/16(xd4)
  [xd5] -> Subsystem1/17(xd5)
  [xd6] -> Subsystem1/18(xd6)
  [xL] -> Subsystem1/19(xL)
  [dX] -> Subsystem1/20(dX)
  [yL] -> Subsystem1/21(yL)
  [dY] -> Subsystem1/22(dY)
  [zL] -> Subsystem1/23(zL)
  [dZ] -> Subsystem1/24(dZ)
  x9/1 -> [x9]
  x5/1 -> [x5]
  x6/1 -> [x6]
  x1/1 -> [x1]
  x4/1 -> [x4]
  x3/1 -> [x3]
  x11/1 -> [x11]
  x10/1 -> [x10]
  x8/1 -> [x8]
  x2/1 -> [x2]
  x7/1 -> [x7]
  x12/1 -> [x12]
  [Phi_d] -> Desired System/1(Phi_d)
  [Theta_d] -> Desired System/2(Theta_d)
  Psi_d/1 -> [Psi_d], Desired System/3(Psi_d)
  " xd"/1 -> Desired System/4(xd)
  yd/1 -> Desired System/5(yd)
  Desired System/2(xd2) -> [xd2]
  Desired System/3(xd3) -> [xd3]
  Desired System/4(xd4) -> [xd4]
  Desired System/5(xd5) -> [xd5]
  Desired System/6(xd6) -> [xd6]
  Desired System/7(xd7) -> [xd7]
  Desired System/8(xd8) -> [xd8]
  Desired System/9(xd9) -> [xd9]
  Desired System/10(xd10) -> [xd10]
  Desired System/11(xd11) -> [xd11]
  Desired System/12(xd12) -> [xd12]
  Desired System/1(xd1) -> [xd1]
  " zd"/1 -> Desired System/6(zd)
  [x1] -> Subsystem1/1(x1)
  [x12] -> Subsystem1/12(x12)
  [x11] -> Subsystem1/11(x11)
  [x10] -> Subsystem1/10(x10)
  [x9] -> Subsystem1/9(x9)
  [x8] -> Subsystem1/8(x8)
  [x7] -> Subsystem1/7(x7)
  [x6] -> Subsystem1/6(x6)
  [x5] -> Subsystem1/5(x5)
  [x4] -> Subsystem1/4(x4)
  [x3] -> Subsystem1/3(x3)
  [x2] -> Subsystem1/2(x2)
  Subsystem1/1(S2) -> "S2 "/1, [S2]
  Subsystem1/2(S4) -> S4/1, [S4]
  Subsystem1/3(S6) -> S6/1, [S6]
  Subsystem1/4(S8) -> S8/1, [S8]
  Subsystem1/5(S10) -> S10/1, [S10]
  Subsystem1/6(S12) -> S12/1, [S12]
  [U1] -> Omega Equations/1(U1)
  [U4] -> Omega Equations/4(U4)
  [U3] -> Omega Equations/3(U3)
  [U2] -> Omega Equations/2(U2)
  Step/1 -> [Theta_d], [Phi_d]
  Mux3/1 -> " Phi_d & Phi"/1
  Mux1/1 -> " Theta_d & Theta"/1
  [Phi_d] -> Mux3/1
  [Theta_d] -> Mux1/1
  [x1] -> Mux3/2
  [x3] -> Mux1/2
  Mux2/1 -> Psi_d & Psi/1
  [Psi_d] -> Mux2/1
  [x5] -> Mux2/2
  Demux/1 -> [xL]
  Demux/2 -> [yL]
  Demux/3 -> [zL]
  Demux1/2 -> [dY]
  Demux1/3 -> [dZ]
  Demux1/1 -> [dX]
  xLeader/1 -> Demux/1
  Distance_d/1 -> Demux1/1
  [x2] -> Subsystem4/2(x2)
  [O] -> Subsystem4/8(Omega)
  [x6] -> Subsystem4/4(x6)
  [xd4] -> Subsystem8/6(xd4)
  [xd2] -> Subsystem4/6(xd2)
  [x3] -> Subsystem8/1(x3)
  Subsystem8/1(U3) -> [U3], U3/1
  Subsystem4/1(U2) -> U2/1, [U2]
  [x1] -> Subsystem4/1(x1)
  [x5] -> Subsystem5/1(x5)
  [O] -> Subsystem8/8(Omega)
  [x6] -> Subsystem5/4(x6)
  [S2] -> Subsystem4/7(S2)
  [xd3] -> Subsystem8/5(xd3)
  [S6] -> Subsystem5/7(S6)
  [xd1] -> Subsystem4/5(xd1)
  Subsystem5/1(U4) -> [U4], U4/1
  [x2] -> Subsystem5/2(x2)
  [x6] -> Subsystem8/4(x6)
  [xd6] -> Subsystem5/6(xd6)
  [x2] -> Subsystem8/2(x2)
  [S4] -> Subsystem8/7(S4)
  [x4] -> Subsystem8/3(x4)
  [xd5] -> Subsystem5/5(xd5)
  [x4] -> Subsystem4/3(x4)
  [x4] -> Subsystem5/3(x4)
  Subsystem10/1(U1) -> [U1], U1/1
  [x12] -> Subsystem10/4(x12)
  [x11] -> Subsystem10/3(x11)
  [dZ] -> Subsystem10/6(dZ)
  [S12] -> Subsystem10/7(S12)
  Subsystem6/1(Ux) -> [Ux], Ux/1
  [x1] -> Subsystem10/1(x1)
  [dX] -> Subsystem6/5(dX)
  [zL] -> Subsystem10/5(zL)
  [S8] -> Subsystem6/6(S8)
  [xL] -> Subsystem6/4(xL)
  [x8] -> Subsystem6/3(x8)
  [x7] -> Subsystem6/2(x7)
  [x3] -> Subsystem10/2(x3)
  [U1] -> Subsystem6/1(U1)
  Subsystem2/1(Uy) -> [Uy], Uy/1
  [U1] -> Subsystem2/1(U1)
  [x10] -> Subsystem2/3(x10)
  [yL] -> Subsystem2/4(yL)
  [S10] -> Subsystem2/6(S10)
  [dY] -> Subsystem2/5(dY)
  [x9] -> Subsystem2/2(x9)

== system RobustFormationControl_IntegerModel_under_Dis/Integer Leader and four followers/Follower 2 System/Follower 2 Quadrotor Model/Quadrotor Dynamic System ==
  U1 : Inport
  U2 : Inport  Port=2
  U3 : Inport  Port=3
  U4 : Inport  Port=4
  Ux : Inport  Port=5
  Uy : Inport  Port=6
  Omega : Inport  Port=7
  Rotational System : Subsystem
  Translational System : Subsystem
  x = x7 : Outport  VectorParamsAs1DForOutWhenUnconnected=off
  y = x9 : Outport  Port=2  VectorParamsAs1DForOutWhenUnconnected=off
  z = x11 : Outport  Port=3  VectorParamsAs1DForOutWhenUnconnected=off
  Phi : Outport  Port=4  VectorParamsAs1DForOutWhenUnconnected=off
  Theta : Outport  Port=5  VectorParamsAs1DForOutWhenUnconnected=off
  Psi : Outport  Port=6  VectorParamsAs1DForOutWhenUnconnected=off
  x2 : Outport  Port=7  VectorParamsAs1DForOutWhenUnconnected=off
  x4 : Outport  Port=8  VectorParamsAs1DForOutWhenUnconnected=off
  x6 : Outport  Port=9  VectorParamsAs1DForOutWhenUnconnected=off
  xdot = x8 : Outport  Port=10  VectorParamsAs1DForOutWhenUnconnected=off
  ydot = x10 : Outport  Port=11  VectorParamsAs1DForOutWhenUnconnected=off
  zdot = x12 : Outport  Port=12  VectorParamsAs1DForOutWhenUnconnected=off
  wires:
  Rotational System/2(Theta or x3) -> Translational System/5(x3), Theta/1  "Theta"
  Rotational System/1(Phi or x1) -> Translational System/4(x1), Phi/1  "Phi"
  U4/1 -> Rotational System/3(U4)
  U2/1 -> Rotational System/1(U2)
  U3/1 -> Rotational System/2(U3)
  Rotational System/3(Psi or x5) -> Psi/1  "Psi"
  Translational System/3(z or x11) -> z = x11/1  "Z"
  Omega/1 -> Rotational System/4(Omega)
  U1/1 -> Translational System/1(U1)
  Translational System/2(y or x9) -> y = x9/1  "Y"
  Translational System/1(x or x7) -> x = x7/1  "X"
  Ux/1 -> Translational System/2(Ux)
  Uy/1 -> Translational System/3(Uy)
  Translational System/4(xdot or x8) -> xdot = x8/1
  Translational System/5(ydot or x10) -> ydot = x10/1
  Translational System/6(zdot or x12) -> zdot = x12/1
  Rotational System/4(x2) -> x2/1
  Rotational System/5(x4) -> x4/1
  Rotational System/6(x6) -> x6/1

== system RobustFormationControl_IntegerModel_under_Dis/Integer Leader and four followers/Follower 3 System/Desired Values/Helical Trajectry ==
  t : Inport
  Gain2 : Gain  Gain=0.2
  Step1 : Step  Time=0  SampleTime=0
  Trigonometric Function : Trigonometry
  Trigonometric Function1 : Trigonometry  Operator=cos
  xd : Outport  VectorParamsAs1DForOutWhenUnconnected=off
  yd : Outport  Port=2  VectorParamsAs1DForOutWhenUnconnected=off
  zd : Outport  Port=3  VectorParamsAs1DForOutWhenUnconnected=off
  Psi_d : Outport  Port=4  VectorParamsAs1DForOutWhenUnconnected=off
  wires:
  Trigonometric Function/1 -> yd/1
  Trigonometric Function1/1 -> xd/1
  Step1/1 -> Psi_d/1
  Gain2/1 -> zd/1
  t/1 -> Gain2/1, Trigonometric Function/1, Trigonometric Function1/1

== system RobustFormationControl_IntegerModel_under_Dis/Integer Leader and four followers/Follower 3 System/Desired Values/Helical Trajectry1 ==
  t : Inport
  Gain : Gain  Gain=dis
  Gain1 : Gain  Gain=2*pi/15
  Gain2 : Gain  Gain=1/15
  Gain3 : Gain  Gain=2*pi/15
  Scope : Scope
  Step : Step  Time=0  After=0  SampleTime=0.03
  Step1 : Step  Time=0  SampleTime=0
  Step2 : Step  Time=5  After=0.5  SampleTime=0.03
  Step3 : Step  Time=10  After=0.5  SampleTime=0.03
  Sum : Sum  Inputs=++-
  Sum1 : Sum  Inputs=|++
  Trigonometric Function : Trigonometry  Operator=cos
  Trigonometric Function1 : Trigonometry
  xd : Outport  VectorParamsAs1DForOutWhenUnconnected=off
  yd : Outport  Port=2  VectorParamsAs1DForOutWhenUnconnected=off
  zd : Outport  Port=3  VectorParamsAs1DForOutWhenUnconnected=off
  Psi_d : Outport  Port=4  VectorParamsAs1DForOutWhenUnconnected=off
  wires:
  Gain3/1 -> Trigonometric Function1/1
  Gain1/1 -> Trigonometric Function/1
  Gain/1 -> Sum1/1
  Trigonometric Function/1 -> Sum1/2
  Sum1/1 -> xd/1
  Step3/1 -> Sum/3
  Step2/1 -> Sum/2
  Sum/1 -> Scope/1, Gain/1
  Step/1 -> Sum/1
  Trigonometric Function1/1 -> yd/1
  Step1/1 -> Psi_d/1
  Gain2/1 -> zd/1
  t/1 -> Gain2/1, Gain3/1, Gain1/1

== system RobustFormationControl_IntegerModel_under_Dis/Integer Leader and four followers/Follower 3 System/Desired Values/Step Inputs Trajectry ==
  Step : Step  Time=0  After=3  SampleTime=0
  Step1 : Step  Time=0  After=5  SampleTime=0
  Step2 : Step  Time=0  SampleTime=0
  Step3 : Step  Time=0  After=2  SampleTime=0
  xd : Outport  VectorParamsAs1DForOutWhenUnconnected=off
  yd : Outport  Port=2  VectorParamsAs1DForOutWhenUnconnected=off
  zd : Outport  Port=3  VectorParamsAs1DForOutWhenUnconnected=off
  Psi_d : Outport  Port=4  VectorParamsAs1DForOutWhenUnconnected=off
  wires:
  Step1/1 -> Psi_d/1
  Step/1 -> zd/1
  Step3/1 -> yd/1
  Step2/1 -> xd/1

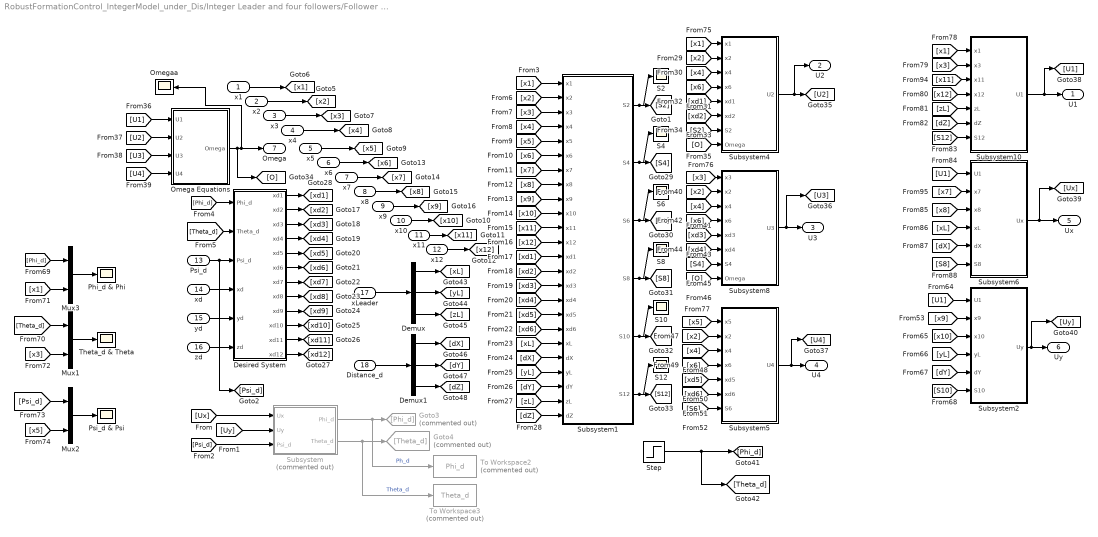
== system RobustFormationControl_IntegerModel_under_Dis/Integer Leader and four followers/Follower 3 System/Follower 2 Quadrotor Model/Control Module1 ==
  x1 : Inport
  x2 : Inport  Port=2
  x3 : Inport  Port=3
  x4 : Inport  Port=4
  x5 : Inport  Port=5
  x6 : Inport  Port=6
  x7 : Inport  Port=7
  x8 : Inport  Port=8
  x9 : Inport  Port=9
  x10 : Inport  Port=10
  x11 : Inport  Port=11
  x12 : Inport  Port=12
  Psi_d : Inport  Port=13
  " xd" : Inport  Port=14
  yd : Inport  Port=15
  " zd" : Inport  Port=16
  xLeader : Inport  Port=17
  Distance_d : Inport  Port=18
  " Phi_d & Phi" : Scope
  " Theta_d & Theta" : Scope
  Demux : Demux  Outputs=3
  Demux1 : Demux  Outputs=3
  Desired System : Subsystem
  Goto3 : Goto  Commented=on  GotoTag=Phi_d
  Goto4 : Goto  Commented=on  GotoTag=Theta_d
  Mux1 : Mux  Inputs=2
  Mux2 : Mux  Inputs=2
  Mux3 : Mux  Inputs=2
  Omega Equations : Subsystem
  Omegaa : Scope
  Psi_d & Psi : Scope
  S{4,6,8,10,12} (5 alike) : Scope
  "S2 " : Scope
  Step : Step  Time=0  After=0.001  SampleTime=0
  Subsystem : Subsystem  Commented=on
  Subsystem1 : Subsystem
  Subsystem10 : Subsystem
  Subsystem2 : Subsystem
  Subsystem4 : Subsystem
  Subsystem5 : Subsystem
  Subsystem6 : Subsystem
  Subsystem8 : Subsystem
  To Workspace2 : ToWorkspace  Commented=on  VariableName=Phi_d  SampleTime=-1
  To Workspace3 : ToWorkspace  Commented=on  VariableName=Theta_d  SampleTime=-1
  U1 : Outport  VectorParamsAs1DForOutWhenUnconnected=off
  U2 : Outport  Port=2  VectorParamsAs1DForOutWhenUnconnected=off
  U3 : Outport  Port=3  VectorParamsAs1DForOutWhenUnconnected=off
  U4 : Outport  Port=4  VectorParamsAs1DForOutWhenUnconnected=off
  Ux : Outport  Port=5  VectorParamsAs1DForOutWhenUnconnected=off
  Uy : Outport  Port=6  VectorParamsAs1DForOutWhenUnconnected=off
  Omega : Outport  Port=7  VectorParamsAs1DForOutWhenUnconnected=off
  wires:
  [x9] -> Subsystem2/2(x9)
  [dY] -> Subsystem2/5(dY)
  [S10] -> Subsystem2/6(S10)
  [yL] -> Subsystem2/4(yL)
  [x10] -> Subsystem2/3(x10)
  [U1] -> Subsystem2/1(U1)
  Subsystem2/1(Uy) -> Uy/1, [Uy]
  [U1] -> Subsystem6/1(U1)
  [x3] -> Subsystem10/2(x3)
  [x7] -> Subsystem6/2(x7)
  [x8] -> Subsystem6/3(x8)
  [xL] -> Subsystem6/4(xL)
  [S8] -> Subsystem6/6(S8)
  [zL] -> Subsystem10/5(zL)
  [dX] -> Subsystem6/5(dX)
  [x1] -> Subsystem10/1(x1)
  Subsystem6/1(Ux) -> Ux/1, [Ux]
  [S12] -> Subsystem10/7(S12)
  [dZ] -> Subsystem10/6(dZ)
  [x11] -> Subsystem10/3(x11)
  [x12] -> Subsystem10/4(x12)
  Subsystem10/1(U1) -> U1/1, [U1]
  [x4] -> Subsystem5/3(x4)
  [x4] -> Subsystem4/3(x4)
  [xd5] -> Subsystem5/5(xd5)
  [x4] -> Subsystem8/3(x4)
  [S4] -> Subsystem8/7(S4)
  [x2] -> Subsystem8/2(x2)
  [xd6] -> Subsystem5/6(xd6)
  [x6] -> Subsystem8/4(x6)
  [x2] -> Subsystem5/2(x2)
  Subsystem5/1(U4) -> U4/1, [U4]
  [xd1] -> Subsystem4/5(xd1)
  [S6] -> Subsystem5/7(S6)
  [xd3] -> Subsystem8/5(xd3)
  [S2] -> Subsystem4/7(S2)
  [x6] -> Subsystem5/4(x6)
  [O] -> Subsystem8/8(Omega)
  [x5] -> Subsystem5/1(x5)
  [x1] -> Subsystem4/1(x1)
  Subsystem4/1(U2) -> [U2], U2/1
  Subsystem8/1(U3) -> U3/1, [U3]
  [x3] -> Subsystem8/1(x3)
  [xd2] -> Subsystem4/6(xd2)
  [xd4] -> Subsystem8/6(xd4)
  [x6] -> Subsystem4/4(x6)
  [O] -> Subsystem4/8(Omega)
  [x2] -> Subsystem4/2(x2)
  Distance_d/1 -> Demux1/1
  xLeader/1 -> Demux/1
  Demux1/1 -> [dX]
  Demux1/3 -> [dZ]
  Demux1/2 -> [dY]
  Demux/3 -> [zL]
  Demux/2 -> [yL]
  Demux/1 -> [xL]
  [x5] -> Mux2/2
  [Psi_d] -> Mux2/1
  Mux2/1 -> Psi_d & Psi/1
  [x3] -> Mux1/2
  [x1] -> Mux3/2
  [Theta_d] -> Mux1/1
  [Phi_d] -> Mux3/1
  Mux1/1 -> " Theta_d & Theta"/1
  Mux3/1 -> " Phi_d & Phi"/1
  Step/1 -> [Phi_d], [Theta_d]
  [U2] -> Omega Equations/2(U2)
  [U3] -> Omega Equations/3(U3)
  [U4] -> Omega Equations/4(U4)
  [U1] -> Omega Equations/1(U1)
  Subsystem1/6(S12) -> [S12], S12/1
  Subsystem1/5(S10) -> [S10], S10/1
  Subsystem1/4(S8) -> [S8], S8/1
  Subsystem1/3(S6) -> [S6], S6/1
  Subsystem1/2(S4) -> [S4], S4/1
  Subsystem1/1(S2) -> [S2], "S2 "/1
  [x2] -> Subsystem1/2(x2)
  [x3] -> Subsystem1/3(x3)
  [x4] -> Subsystem1/4(x4)
  [x5] -> Subsystem1/5(x5)
  [x6] -> Subsystem1/6(x6)
  [x7] -> Subsystem1/7(x7)
  [x8] -> Subsystem1/8(x8)
  [x9] -> Subsystem1/9(x9)
  [x10] -> Subsystem1/10(x10)
  [x11] -> Subsystem1/11(x11)
  [x12] -> Subsystem1/12(x12)
  [x1] -> Subsystem1/1(x1)
  " zd"/1 -> Desired System/6(zd)
  Desired System/1(xd1) -> [xd1]
  Desired System/12(xd12) -> [xd12]
  Desired System/11(xd11) -> [xd11]
  Desired System/10(xd10) -> [xd10]
  Desired System/9(xd9) -> [xd9]
  Desired System/8(xd8) -> [xd8]
  Desired System/7(xd7) -> [xd7]
  Desired System/6(xd6) -> [xd6]
  Desired System/5(xd5) -> [xd5]
  Desired System/4(xd4) -> [xd4]
  Desired System/3(xd3) -> [xd3]
  Desired System/2(xd2) -> [xd2]
  yd/1 -> Desired System/5(yd)
  " xd"/1 -> Desired System/4(xd)
  Psi_d/1 -> Desired System/3(Psi_d), [Psi_d]
  [Theta_d] -> Desired System/2(Theta_d)
  [Phi_d] -> Desired System/1(Phi_d)
  x12/1 -> [x12]
  x7/1 -> [x7]
  x2/1 -> [x2]
  x8/1 -> [x8]
  x10/1 -> [x10]
  x11/1 -> [x11]
  x3/1 -> [x3]
  x4/1 -> [x4]
  x1/1 -> [x1]
  x6/1 -> [x6]
  x5/1 -> [x5]
  x9/1 -> [x9]
  [dZ] -> Subsystem1/24(dZ)
  [zL] -> Subsystem1/23(zL)
  [dY] -> Subsystem1/22(dY)
  [yL] -> Subsystem1/21(yL)
  [dX] -> Subsystem1/20(dX)
  [xL] -> Subsystem1/19(xL)
  [xd6] -> Subsystem1/18(xd6)
  [xd5] -> Subsystem1/17(xd5)
  [xd4] -> Subsystem1/16(xd4)
  [xd3] -> Subsystem1/15(xd3)
  [xd2] -> Subsystem1/14(xd2)
  [xd1] -> Subsystem1/13(xd1)
  Subsystem/2(Theta_d) -> Goto4/1, To Workspace3/1  "Theta_d"
  Subsystem/1(Phi_d) -> Goto3/1, To Workspace2/1  "Ph_d"
  [Psi_d] -> Subsystem/3(Psi_d)
  [Uy] -> Subsystem/2(Uy)
  [Ux] -> Subsystem/1(Ux)
  Omega Equations/1(Omega) -> Omega/1, Omegaa/1, [O]
